simulink model "03_matlab_landslide"  (R2026a)
settings: Solver=VariableStepAuto  StopTime=60
settings Model: PacingRate=10  Creator=Arosh rolly  LastModifiedBy=Arosh rolly

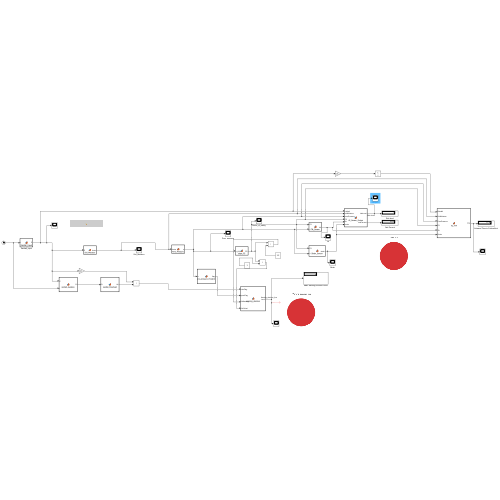
[thumbnail: Simulink's stored preview of the top-level diagram]
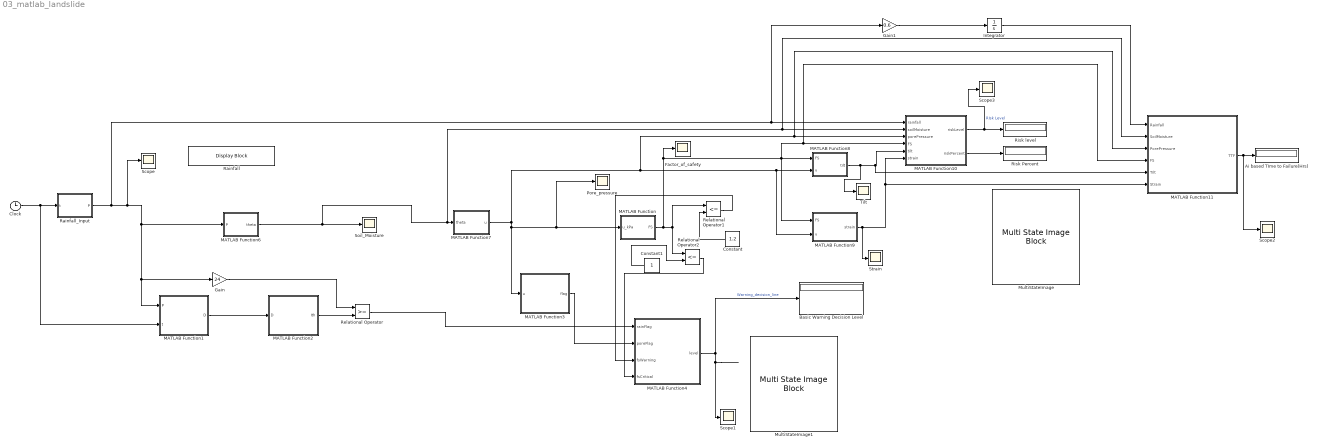
== system 03_matlab_landslide ==
  Ai based TIme to Failure(Hrs) : Display
  Basic Warning Decision Level : Display
  Clock : Clock
  Constant : Constant  Value=1.2
  Constant1 : Constant
  Factor_of_safety : Scope
      settings: ActiveDisplayYMinimum=0.67876373507093857  ActiveDisplayYMaximum=1.520701331107178  DataLoggingVariableName=ScopeData3
  Gain : Gain  Gain=24
  Gain1 : Gain  Gain=0.6
  Integrator : Integrator
  MATLAB Function : MATLAB Function  TreatAsAtomicUnit=on
  MATLAB Function1 : MATLAB Function  TreatAsAtomicUnit=on
  MATLAB Function10 : MATLAB Function  TreatAsAtomicUnit=on
  MATLAB Function11 : MATLAB Function  TreatAsAtomicUnit=on
  MATLAB Function2 : MATLAB Function  TreatAsAtomicUnit=on
  MATLAB Function3 : MATLAB Function  TreatAsAtomicUnit=on
  MATLAB Function4 : MATLAB Function  TreatAsAtomicUnit=on
  MATLAB Function6 : MATLAB Function  TreatAsAtomicUnit=on
  MATLAB Function7 : MATLAB Function  TreatAsAtomicUnit=on
  MATLAB Function8 : MATLAB Function  TreatAsAtomicUnit=on
  MATLAB Function9 : MATLAB Function  TreatAsAtomicUnit=on
  MultiStateImage : MultiStateImageBlock
  MultiStateImage1 : MultiStateImageBlock
  Pore_pressure : Scope
      settings: ActiveDisplayYMinimum=-2.905798457705417  ActiveDisplayYMaximum=29.116186119348761  DataLoggingVariableName=ScopeData2
  Rainfall : DisplayBlock  LabelPosition=Hide  Transparency=1  GridColor=[0.502, 0.502, 0.502]
  Rainfall_Input : MATLAB Function  TreatAsAtomicUnit=on
  Relational Operator : RelationalOperator  OutDataTypeStr=boolean  RndMeth=Simplest  InputSameDT=off
  Relational Operator1 : RelationalOperator  Operator=<=  OutDataTypeStr=boolean  RndMeth=Simplest  InputSameDT=off
  Relational Operator2 : RelationalOperator  Operator=<=  OutDataTypeStr=boolean  RndMeth=Simplest  InputSameDT=off
  Risk Percent : Display
  Risk level : Display
  Scope{,1..3} (4 alike) : Scope
      Scope settings: ActiveDisplayYMinimum=-31.476873124504095  ActiveDisplayYMaximum=244.67576835273502
      Scope1 settings: ActiveDisplayYMinimum=0.62500000000000011  ActiveDisplayYMaximum=4.375  DataLoggingVariableName=ScopeData6
      Scope2 settings: ActiveDisplayYMinimum=9.6742834573922849  ActiveDisplayYMaximum=31.791685658907735  DataLoggingVariableName=ScopeData7
      Scope3 settings: ActiveDisplayYMinimum=0.62500000000000011  ActiveDisplayYMaximum=4.375  DataLoggingVariableName=ScopeData8
  Soil_Moisture : Scope
      settings: ActiveDisplayYMinimum=0.12729290208419816  ActiveDisplayYMaximum=1.0969674553239779
  Strain : Scope
      settings: ActiveDisplayYMinimum=-0.054696719481509185  ActiveDisplayYMaximum=0.59244831533358266  DataLoggingVariableName=ScopeData5
  Tilt : Scope
      settings: ActiveDisplayYMinimum=-0.068591730340824664  ActiveDisplayYMaximum=1.1182147730674223  DataLoggingVariableName=ScopeData4
  wires:
  Rainfall_Input/1(P) -> Gain1/1, MATLAB Function10/1(rainfall), Scope/1, MATLAB Function6/1(P), MATLAB Function1/1(P), Gain/1
  MATLAB Function1/1(D) -> MATLAB Function2/1(D)
  MATLAB Function2/1(Ith) -> Relational Operator/2
  MATLAB Function/1(FS) -> MATLAB Function11/4(FS), MATLAB Function10/4(FS), MATLAB Function9/1(FS), MATLAB Function8/1(FS), Factor_of_safety/1, Relational Operator2/1, Relational Operator1/1
  Constant/1 -> Relational Operator1/2
  Constant1/1 -> Relational Operator2/2
  Relational Operator/1 -> MATLAB Function4/1(rainFlag)
  MATLAB Function3/1(flag) -> MATLAB Function4/2(poreFlag)
  Relational Operator1/1 -> MATLAB Function4/3(fsWarning)
  Relational Operator2/1 -> MATLAB Function4/4(fsCritical)
  MATLAB Function4/1(level) -> Scope1/1, Basic Warning Decision Level/1  "Warning_decision_line"
  MATLAB Function6/1(theta) -> MATLAB Function11/2(SoilMoisture), MATLAB Function10/2(soilMoisture), MATLAB Function7/1(theta), Soil_Moisture/1
  MATLAB Function7/1(u) -> Pore_pressure/1, MATLAB Function/1(u_kPa), MATLAB Function3/1(u), MATLAB Function10/3(porePressure), MATLAB Function11/3(PorePressure), MATLAB Function9/2(u), MATLAB Function8/2(u)
  Clock/1 -> MATLAB Function1/2(t), Rainfall_Input/1(t)
  Gain/1 -> Relational Operator/1
  MATLAB Function8/1(tilt) -> Tilt/1, MATLAB Function11/5(Tilt), MATLAB Function10/5(tilt)
  MATLAB Function9/1(strain) -> MATLAB Function11/6(Strain), MATLAB Function10/6(strain), Strain/1
  MATLAB Function10/2(riskPercent) -> Risk Percent/1
  MATLAB Function10/1(riskLevel) -> Scope3/1, Risk level/1  "RIsk Level"
  Gain1/1 -> Integrator/1
  Integrator/1 -> MATLAB Function11/1(Rainfall)
  MATLAB Function11/1(TTF) -> Scope2/1, Ai based TIme to Failure(Hrs)/1

== matlab function 03_matlab_landslide/MATLAB Function11 ==
  data: Rainfall input; TTF output; SoilMoisture input; PorePressure input; FS input; Tilt input; Strain input
function TTF = AI_TTF(Rainfall, SoilMoisture, PorePressure, FS, Tilt, Strain)
%#codegen
% AI Time-To-Failure estimator
% Munnar / Idukki landslide model
%
% OUTPUT:
% TTF = Estimated remaining time to failure in hours

%% Reference values from the supplied Munnar/Idukki database

% Rainfall
Rain_min = 0;
Rain_max = 450;

% Soil moisture
Moist_min = 18.0;
Moist_max = 58.4;

% Pore pressure
Pore_min = -15.0;
Pore_max = 41.0;

% Factor of Safety
FS_safe = 1.85;
FS_failure = 0.99;

% Surface tilt
Tilt_min = 0.02;
Tilt_max = 4.80;

% Shear strain
Strain_min = 12;
Strain_max = 2850;

%% Normalize sensor values

Rain_score = (Rainfall - Rain_min) / ...
             (Rain_max - Rain_min);

Moist_score = (SoilMoisture - Moist_min) / ...
              (Moist_max - Moist_min);

Pore_score = (PorePressure - Pore_min) / ...
             (Pore_max - Pore_min);

% Lower FS means greater danger
FS_score = (FS_safe - FS) / ...
           (FS_safe - FS_failure);

Tilt_score = (Tilt - Tilt_min) / ...
             (Tilt_max - Tilt_min);

Strain_score = (Strain - Strain_min) / ...
               (Strain_max - Strain_min);

%% Limit all scores to 0-1

Rain_score = min(max(Rain_score,0),1);
Moist_score = min(max(Moist_score,0),1);
Pore_score = min(max(Pore_score,0),1);
FS_score = min(max(FS_score,0),1);
Tilt_score = min(max(Tilt_score,0),1);
Strain_score = min(max(Strain_score,0),1);

%% Sensor fusion

% Higher weight is given to FS and strain

Progress = ...
      0.10 * Rain_score ...
    + 0.10 * Moist_score ...
    + 0.10 * Pore_score ...
    + 0.30 * FS_score ...
    + 0.15 * Tilt_score ...
    + 0.25 * Strain_score;

%% Convert progression to TTF

if Progress >= 1.0

    % Failure condition
    TTF = 0;

elseif Progress >= 0.95

    % 1 hour to failure
    TTF = 1.0 - ...
        (Progress - 0.95) * (1.0 - 0.25) / 0.04;

elseif Progress >= 0.85

    % 3 hours to failure
    TTF = 3.0 - ...
        (Progress - 0.85) * (3.0 - 1.0) / 0.10;

elseif Progress >= 0.70

    % 6 hours to failure
    TTF = 6.0 - ...
        (Progress - 0.70) * (6.0 - 3.0) / 0.15;

elseif Progress >= 0.50

    % 12 hours to failure
    TTF = 12.0 - ...
        (Progress - 0.50) * (12.0 - 6.0) / 0.20;

elseif Progress >= 0.25

    % 24 hours to failure
    TTF = 24.0 - ...
        (Progress - 0.25) * (24.0 - 12.0) / 0.25;

else

    % 42 hours to failure
    TTF = 42.0 - ...
        Progress * (42.0 - 24.0) / 0.25;

end

%% Prevent negative values

TTF = max(TTF,0);

end

== matlab function 03_matlab_landslide/MATLAB Function1 ==
  settings: updateMethod=DISCRETE
  data: P input; D output; t input
function D = rainfall_duration(P,t)

% P = rainfall intensity in mm/hour
% t = simulation time in seconds
% 60 simulation seconds = 36 real hours
% D = rainfall duration in days

persistent startTime

if isempty(startTime)
    startTime = -1;
end

if P > 0

    if startTime < 0
        startTime = t;
    end

    % Simulation seconds -> real hours -> days
    D = ((t - startTime) * 0.6) / 24;

else

    startTime = -1;
    D = 0;

end

end

== matlab function 03_matlab_landslide/MATLAB Function ==
  data: u_kPa input; FS output
function FS = slope_FS(u_kPa)

% Convert pore pressure from kPa to Pa
u = u_kPa * 1000;

% Slope parameters
c = 12000;       % Cohesion (Pa)
phi = 28;        % Friction angle (degrees)
gamma = 18000;   % Unit weight (N/m^3)
z = 2.5;         % Soil depth (m)
beta = 32;       % Slope angle (degrees)

% Factor of Safety
numerator = c + (gamma*z*cosd(beta)^2 - u)*tand(phi);

denominator = gamma*z*sind(beta)*cosd(beta);

FS = numerator / denominator;

end

== matlab function 03_matlab_landslide/MATLAB Function2 ==
  data: D input; Ith output
function Ith = rainfall_threshold(D)

% Rainfall threshold in mm/day

if D <= 0
    Ith = 1e6;
else
    Ith = 43.26 * D^(-0.78);
end

end

== matlab function 03_matlab_landslide/MATLAB Function3 ==
  data: u input; flag output
function flag = pore_pressure_threshold(u)

u_threshold = 20;   % Pa

if u >= u_threshold
    flag = 1;
else
    flag = 0;
end

== matlab function 03_matlab_landslide/MATLAB Function4 ==
  data: rainFlag input; level output; poreFlag input; fsWarning input; fsCritical input
function level = warning_decision(rainFlag,poreFlag,fsWarning,fsCritical)

if fsCritical == 1
    level = 4;          % RED - CRITICAL
elseif fsWarning == 1
    level = 3;          % ORANGE - HIGH WARNING
elseif poreFlag == 1 || rainFlag == 1
    level = 2;          % YELLOW - WARNING
else
    level = 1;          % GREEN - SAFE
end

end

== matlab function 03_matlab_landslide/Rainfall_Input ==
  data: t input; P output
function P = Rainfall_Input(t)

% t = simulation time in seconds
% 60 simulation seconds represents 36 hours
% P = rainfall intensity in mm/hour

% Convert simulation time to equivalent real time
time_hr = t * 0.6;

if time_hr < 6
    P = 0;
elseif time_hr < 12
    P = 10;
elseif time_hr < 18
    P = 25;
elseif time_hr < 24
    P = 40;
elseif time_hr < 36
    P = 20;
else
    P = 0;
end

end

== matlab function 03_matlab_landslide/MATLAB Function6 ==
  settings: updateMethod=DISCRETE
  data: P input; theta output
function theta = Soil_Moisture(P)

% P = rainfall intensity (mm/hour)
% theta = normalized soil moisture (0 to 1)

Ki = 0.004;
Kd = 0.02;

% 1 simulation second = 0.6 real hours
Ts = 0.6;

theta0 = 0.25;

persistent theta_prev

if isempty(theta_prev)
    theta_prev = theta0;
end

theta = theta_prev + Ts*(Ki*P - Kd*theta_prev);

theta = min(max(theta,0),1);

theta_prev = theta;

end

== matlab function 03_matlab_landslide/MATLAB Function7 ==
  data: theta input; u output
function u = Pore_Pressure(theta)

% theta = soil moisture
% u = pore pressure in kPa

Ku = 2;
Kdr = 0.05;

% 1 simulation second = 0.6 real hours
Ts = 0.6;

persistent u_prev

if isempty(u_prev)
    u_prev = 0;
end

u = u_prev + Ts*(Ku*theta - Kdr*u_prev);

u = max(u,0);

u_prev = u;

end

== matlab function 03_matlab_landslide/MATLAB Function8 ==
  data: FS input; u input; tilt output
function tilt = Tilt_Sensor(FS,u)

% Simulated tilt sensor
% Output: tilt angle in degrees

persistent tilt_prev

if isempty(tilt_prev)
    tilt_prev = 0.05;
end

% Small natural/background movement
baseTilt = 0.05;

% Tilt increases as FS decreases
instability = max(0,1.2-FS);

% Additional influence of pore pressure
pressureEffect = 0.002*u;

targetTilt = baseTilt + ...
             2.5*instability + ...
             pressureEffect;

% Smooth sensor response
alpha = 0.15;

tilt = tilt_prev + alpha*(targetTilt-tilt_prev);

tilt_prev = tilt;

end

== matlab function 03_matlab_landslide/MATLAB Function9 ==
  data: FS input; u input; strain output
function strain = Strain_Sensor(FS,u)

% Simulated strain sensor
% Output: strain in percent

persistent strain_prev

if isempty(strain_prev)
    strain_prev = 0.01;
end

% Stable baseline strain
baseStrain = 0.01;

% Instability component
instability = max(0,1.2-FS);

% Pore-pressure influence
pressureEffect = 0.0005*u;

targetStrain = baseStrain + ...
               1.5*instability + ...
               pressureEffect;

% Smooth sensor response
alpha = 0.12;

strain = strain_prev + ...
         alpha*(targetStrain-strain_prev);

strain_prev = strain;

end

== matlab function 03_matlab_landslide/MATLAB Function10 ==
  data: rainfall input; soilMoisture input; porePressure input; FS input; riskLevel output; tilt input; strain input; riskPercent output
function [riskLevel, riskPercent] = AI_Sensor_Fusion( ...
    rainfall, soilMoisture, porePressure, FS, tilt, strain)

% AI SENSOR FUSION - Munnar/Idukki Landslide Warning System
%
% Inputs:
% rainfall     = cumulative rainfall (mm)
% soilMoisture = volumetric soil moisture (%)
% porePressure = pore water pressure (kPa)
% FS           = factor of safety
% tilt         = surface tilt angle (degrees)
% strain       = subsurface shear strain (microstrain)
%
% Outputs:
% riskLevel    = 1 Safe     -> GREEN
%                2 Warning  -> YELLOW
%                3 High     -> ORANGE
%                4 Critical -> RED
%
% riskPercent  = fused risk score (0-100 %)

%% ---------------------------------------------------------
% 1. Normalize the six sensor parameters
% ---------------------------------------------------------

% Rainfall: 0 to 340 mm
rainScore = rainfall / 340;

% Soil moisture: 18 to 58 %
moistureScore = (soilMoisture - 18) / (58 - 18);

% Pore pressure: -15 to +38 kPa
poreScore = (porePressure + 15) / (38 + 15);

% Factor of Safety:
% Higher FS = safer, therefore invert it.
FSscore = (1.85 - FS) / (1.85 - 0.98);

% Surface tilt: 0.02 to 2.10 degrees
tiltScore = (tilt - 0.02) / (2.10 - 0.02);

% Shear strain: 12 to 2850 microstrain
strainScore = (strain - 12) / (2850 - 12);

%% ---------------------------------------------------------
% 2. Limit normalized values to 0-1
% ---------------------------------------------------------

rainScore     = min(max(rainScore,0),1);
moistureScore = min(max(moistureScore,0),1);
poreScore     = min(max(poreScore,0),1);
FSscore       = min(max(FSscore,0),1);
tiltScore     = min(max(tiltScore,0),1);
strainScore   = min(max(strainScore,0),1);

%% ---------------------------------------------------------
% 3. AI Sensor Fusion
% ---------------------------------------------------------

riskScore = ...
      0.15 * rainScore ...
    + 0.15 * moistureScore ...
    + 0.15 * poreScore ...
    + 0.25 * FSscore ...
    + 0.15 * tiltScore ...
    + 0.15 * strainScore;

%% ---------------------------------------------------------
% 4. Convert fused score to percentage
% ---------------------------------------------------------

riskPercent = riskScore * 100;

%% ---------------------------------------------------------
% 5. Determine warning level
% ---------------------------------------------------------

if FS <= 0.98 || strain >= 2850 || tilt >= 2.10

    riskLevel = 4;       % RED - CRITICAL

elseif FS <= 1.15 || strain >= 420 || tilt >= 0.35

    riskLevel = 3;       % ORANGE - HIGH WARNING

elseif FS <= 1.42 || strain >= 85 || tilt >= 0.08

    riskLevel = 2;       % YELLOW - WARNING

else

    riskLevel = 1;       % GREEN - SAFE

end

end
